simulink model "LSC_Integration"  (R2022b)
settings: Solver=FixedStepDiscrete  StartTime=0.0  StopTime=130  FixedStep=Ts  RelTol=1e-3
values from neighbouring files (symbols this model uses):
  LUX_AHB = 50    [build_B3_AHB.m]
  LUX_OFF = 2000    [build_B2_AutoHeadlamp.m]
  LUX_ON = 1000    [build_B2_AutoHeadlamp.m]
  T_OFF = 5    [build_B2_AutoHeadlamp.m]
  T_ON = 2    [build_B2_AutoHeadlamp.m]
  T_REARM = 2    [build_B3_AHB.m]
  T_TUNNEL = 0.3    [build_B2_AutoHeadlamp.m]
  Ts = 0.01    [build_B2_AutoHeadlamp.m]    (also in build_B3_AHB.m)
  V_AHB_OFF = 30    [build_B3_AHB.m]
  V_AHB_ON = 40    [build_B3_AHB.m]
undefined symbols (not defined in the file or in its folder): A_ESS_OFF, A_ESS_ON, F_BLINK, F_ESS, F_HYPER, I_NOM, LUX_MAX, N_COMFORT, POS_DIM, R_OPEN, R_SHORT, T_ABSENT, T_ARM, T_CONF, T_DEB, T_FMH, T_FMH_MAX, T_FMH_STEP, T_HEAL, T_INRUSH, T_RECOVER, T_SHORT, T_SOFT, TAIL_DIM, TAU_LUX, U_BAT_MIN, V_EFF, V_ESS, V_RESUME
libraries: simulink x1
settings Model: Creator=LENOVO  LastModifiedBy=LENOVO

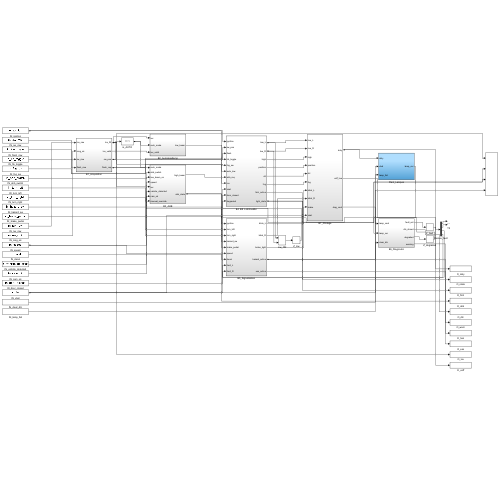
[thumbnail: Simulink's stored preview of the top-level diagram]
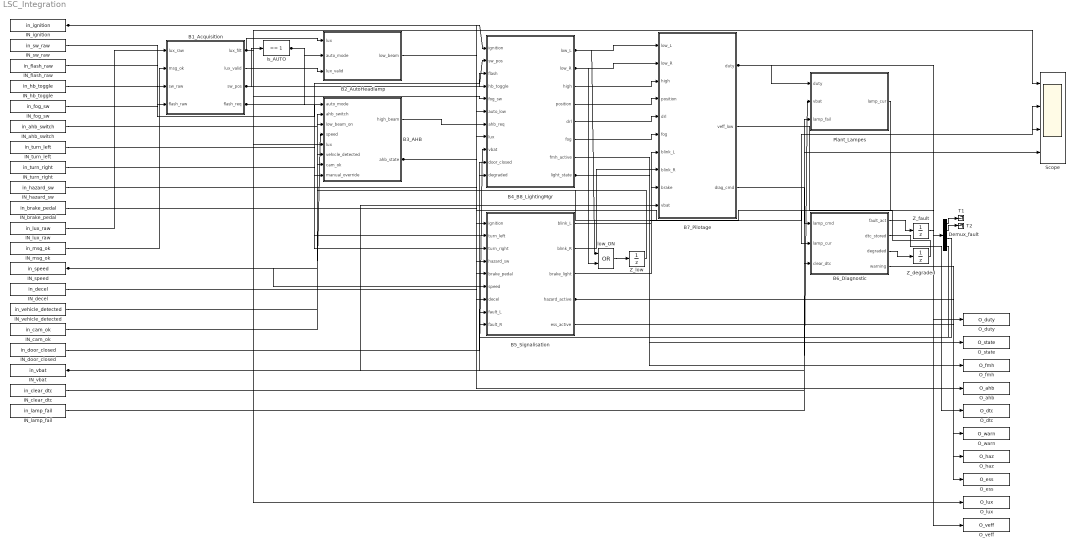
== system LSC_Integration ==
  B1_Acquisition : Subsystem
  B2_AutoHeadlamp : Subsystem
  B3_AHB : Subsystem
  B4_B8_LightingMgr : Subsystem
  B5_Signalisation : Subsystem
  B6_Diagnostic : Subsystem
  B7_Pilotage : Subsystem
  Demux_fault : Demux
  IN_ahb_switch : FromWorkspace  VariableName=in_ahb_switch  SampleTime=Ts  Interpolate=off  OutputAfterFinalValue=Holding final value
  IN_brake_pedal : FromWorkspace  VariableName=in_brake_pedal  SampleTime=Ts  Interpolate=off  OutputAfterFinalValue=Holding final value
  IN_cam_ok : FromWorkspace  VariableName=in_cam_ok  SampleTime=Ts  Interpolate=off  OutputAfterFinalValue=Holding final value
  IN_clear_dtc : FromWorkspace  VariableName=in_clear_dtc  SampleTime=Ts  Interpolate=off  OutputAfterFinalValue=Holding final value
  IN_decel : FromWorkspace  VariableName=in_decel  SampleTime=Ts  OutputAfterFinalValue=Holding final value
  IN_door_closed : FromWorkspace  VariableName=in_door_closed  SampleTime=Ts  Interpolate=off  OutputAfterFinalValue=Holding final value
  IN_flash_raw : FromWorkspace  VariableName=in_flash_raw  SampleTime=Ts  Interpolate=off  OutputAfterFinalValue=Holding final value
  IN_fog_sw : FromWorkspace  VariableName=in_fog_sw  SampleTime=Ts  Interpolate=off  OutputAfterFinalValue=Holding final value
  IN_hazard_sw : FromWorkspace  VariableName=in_hazard_sw  SampleTime=Ts  Interpolate=off  OutputAfterFinalValue=Holding final value
  IN_hb_toggle : FromWorkspace  VariableName=in_hb_toggle  SampleTime=Ts  Interpolate=off  OutputAfterFinalValue=Holding final value
  IN_ignition : FromWorkspace  VariableName=in_ignition  SampleTime=Ts  Interpolate=off  OutputAfterFinalValue=Holding final value
  IN_lamp_fail : FromWorkspace  VariableName=in_lamp_fail  SampleTime=Ts  Interpolate=off  OutputAfterFinalValue=Holding final value
  IN_lux_raw : FromWorkspace  VariableName=in_lux_raw  SampleTime=Ts  OutputAfterFinalValue=Holding final value
  IN_msg_ok : FromWorkspace  VariableName=in_msg_ok  SampleTime=Ts  Interpolate=off  OutputAfterFinalValue=Holding final value
  IN_speed : FromWorkspace  VariableName=in_speed  SampleTime=Ts  OutputAfterFinalValue=Holding final value
  IN_sw_raw : FromWorkspace  VariableName=in_sw_raw  SampleTime=Ts  Interpolate=off  OutputAfterFinalValue=Holding final value
  IN_turn_left : FromWorkspace  VariableName=in_turn_left  SampleTime=Ts  Interpolate=off  OutputAfterFinalValue=Holding final value
  IN_turn_right : FromWorkspace  VariableName=in_turn_right  SampleTime=Ts  Interpolate=off  OutputAfterFinalValue=Holding final value
  IN_vbat : FromWorkspace  VariableName=in_vbat  SampleTime=Ts  OutputAfterFinalValue=Holding final value
  IN_vehicle_detected : FromWorkspace  VariableName=in_vehicle_detected  SampleTime=Ts  Interpolate=off  OutputAfterFinalValue=Holding final value
  O_ahb : ToWorkspace  VariableName=O_ahb  SaveFormat=Timeseries  SampleTime=-1
  O_dtc : ToWorkspace  VariableName=O_dtc  SaveFormat=Timeseries  SampleTime=-1
  O_duty : ToWorkspace  VariableName=O_duty  SaveFormat=Timeseries  SampleTime=-1
  O_ess : ToWorkspace  VariableName=O_ess  SaveFormat=Timeseries  SampleTime=-1
  O_fmh : ToWorkspace  VariableName=O_fmh  SaveFormat=Timeseries  SampleTime=-1
  O_haz : ToWorkspace  VariableName=O_haz  SaveFormat=Timeseries  SampleTime=-1
  O_lux : ToWorkspace  VariableName=O_lux  SaveFormat=Timeseries  SampleTime=-1
  O_state : ToWorkspace  VariableName=O_state  SaveFormat=Timeseries  SampleTime=-1
  O_veff : ToWorkspace  VariableName=O_veff  SaveFormat=Timeseries  SampleTime=-1
  O_warn : ToWorkspace  VariableName=O_warn  SaveFormat=Timeseries  SampleTime=-1
  Plant_Lampes : Subsystem
  Scope : Scope  NumInputPorts=4
  T1 : Terminator
  T2 : Terminator
  Z_degraded : UnitDelay  SampleTime=Ts  HasFrameUpgradeWarning=on
  Z_fault : UnitDelay  SampleTime=Ts  HasFrameUpgradeWarning=on
  Z_low : UnitDelay  SampleTime=Ts  HasFrameUpgradeWarning=on
  is_AUTO : simulink/Logic and Bit Operations/Compare To Constant  relop===  const=1  OutDataTypeStr=boolean
  low_ON : Logic  Operator=OR  AllPortsSameDT=off  OutDataTypeStr=boolean
  wires:
  IN_lux_raw/1 -> B1_Acquisition/1(lux_raw)
  IN_msg_ok/1 -> B1_Acquisition/2(msg_ok)
  IN_sw_raw/1 -> B1_Acquisition/3(sw_raw)
  IN_flash_raw/1 -> B1_Acquisition/4(flash_raw)
  B1_Acquisition/3(sw_pos) -> is_AUTO/1, B4_B8_LightingMgr/2(sw_pos)
  B1_Acquisition/1(lux_filt) -> B2_AutoHeadlamp/1(lux), B3_AHB/5(lux), B4_B8_LightingMgr/8(lux), O_lux/1, Scope/1
  is_AUTO/1 -> B2_AutoHeadlamp/2(auto_mode), B3_AHB/1(auto_mode)
  B1_Acquisition/2(lux_valid) -> B2_AutoHeadlamp/3(lux_valid)
  IN_ahb_switch/1 -> B3_AHB/2(ahb_switch)
  Z_low/1 -> B3_AHB/3(low_beam_on)
  IN_speed/1 -> B3_AHB/4(speed), B5_Signalisation/6(speed)
  IN_vehicle_detected/1 -> B3_AHB/6(vehicle_detected)
  IN_cam_ok/1 -> B3_AHB/7(cam_ok)
  B1_Acquisition/4(flash_req) -> B3_AHB/8(manual_override), B4_B8_LightingMgr/3(flash)
  IN_ignition/1 -> B4_B8_LightingMgr/1(ignition), B5_Signalisation/1(ignition)
  IN_hb_toggle/1 -> B4_B8_LightingMgr/4(hb_toggle)
  IN_fog_sw/1 -> B4_B8_LightingMgr/5(fog_sw)
  B2_AutoHeadlamp/1(low_beam) -> B4_B8_LightingMgr/6(auto_low)
  B3_AHB/1(high_beam) -> B4_B8_LightingMgr/7(ahb_req)
  IN_vbat/1 -> B4_B8_LightingMgr/9(vbat), B7_Pilotage/10(vbat), Plant_Lampes/2(vbat)
  IN_door_closed/1 -> B4_B8_LightingMgr/10(door_closed)
  Z_degraded/1 -> B4_B8_LightingMgr/11(degraded)
  B4_B8_LightingMgr/1(low_L) -> low_ON/1, B7_Pilotage/1(low_L)
  B4_B8_LightingMgr/2(low_R) -> low_ON/2, B7_Pilotage/2(low_R)
  low_ON/1 -> Z_low/1
  IN_turn_left/1 -> B5_Signalisation/2(turn_left)
  IN_turn_right/1 -> B5_Signalisation/3(turn_right)
  IN_hazard_sw/1 -> B5_Signalisation/4(hazard_sw)
  IN_brake_pedal/1 -> B5_Signalisation/5(brake_pedal)
  IN_decel/1 -> B5_Signalisation/7(decel)
  Demux_fault/3 -> B5_Signalisation/8(fault_L)
  Demux_fault/4 -> B5_Signalisation/9(fault_R)
  Demux_fault/1 -> T1/1
  Demux_fault/2 -> T2/1
  B4_B8_LightingMgr/3(high) -> B7_Pilotage/3(high)
  B4_B8_LightingMgr/4(position) -> B7_Pilotage/4(position)
  B4_B8_LightingMgr/5(drl) -> B7_Pilotage/5(drl)
  B4_B8_LightingMgr/6(fog) -> B7_Pilotage/6(fog)
  B5_Signalisation/1(blink_L) -> B7_Pilotage/7(blink_L)
  B5_Signalisation/2(blink_R) -> B7_Pilotage/8(blink_R)
  B5_Signalisation/3(brake_light) -> B7_Pilotage/9(brake)
  B7_Pilotage/1(duty) -> Plant_Lampes/1(duty), O_duty/1
  IN_lamp_fail/1 -> Plant_Lampes/3(lamp_fail)
  B7_Pilotage/3(diag_cmd) -> B6_Diagnostic/1(lamp_cmd)
  Plant_Lampes/1(lamp_cur) -> B6_Diagnostic/2(lamp_cur)
  IN_clear_dtc/1 -> B6_Diagnostic/3(clear_dtc)
  B6_Diagnostic/1(fault_act) -> Z_fault/1
  Z_fault/1 -> Demux_fault/1
  B6_Diagnostic/3(degraded) -> Z_degraded/1
  B4_B8_LightingMgr/8(light_state) -> O_state/1, Scope/2
  B4_B8_LightingMgr/7(fmh_active) -> O_fmh/1
  B3_AHB/2(ahb_state) -> O_ahb/1, Scope/3
  B6_Diagnostic/2(dtc_stored) -> O_dtc/1
  B6_Diagnostic/4(warning) -> O_warn/1
  B5_Signalisation/4(hazard_active) -> O_haz/1, Scope/4
  B5_Signalisation/5(ess_active) -> O_ess/1
  B7_Pilotage/2(veff_low) -> O_veff/1

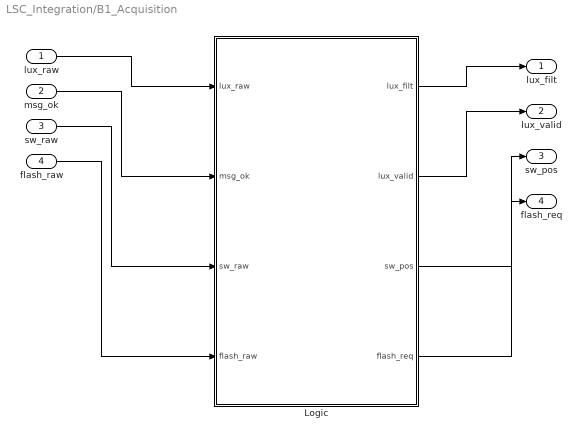
== system LSC_Integration/B1_Acquisition ==
  lux_raw : Inport
  msg_ok : Inport  Port=2
  sw_raw : Inport  Port=3
  flash_raw : Inport  Port=4
  Logic : MATLAB Function  TreatAsAtomicUnit=on
  lux_filt : Outport
  lux_valid : Outport  Port=2
  sw_pos : Outport  Port=3
  flash_req : Outport  Port=4
  wires:
  lux_raw/1 -> Logic/1(lux_raw)
  msg_ok/1 -> Logic/2(msg_ok)
  sw_raw/1 -> Logic/3(sw_raw)
  flash_raw/1 -> Logic/4(flash_raw)
  Logic/1(lux_filt) -> lux_filt/1
  Logic/2(lux_valid) -> lux_valid/1
  Logic/3(sw_pos) -> sw_pos/1
  Logic/4(flash_req) -> flash_req/1

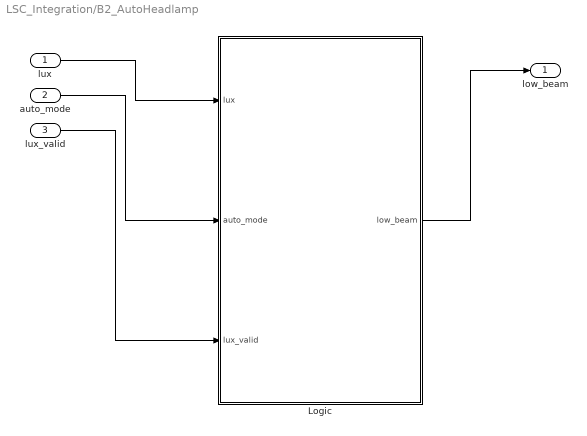
== system LSC_Integration/B2_AutoHeadlamp ==
  lux : Inport
  auto_mode : Inport  Port=2
  lux_valid : Inport  Port=3
  Logic : MATLAB Function  TreatAsAtomicUnit=on
  low_beam : Outport
  wires:
  lux/1 -> Logic/1(lux)
  auto_mode/1 -> Logic/2(auto_mode)
  lux_valid/1 -> Logic/3(lux_valid)
  Logic/1(low_beam) -> low_beam/1

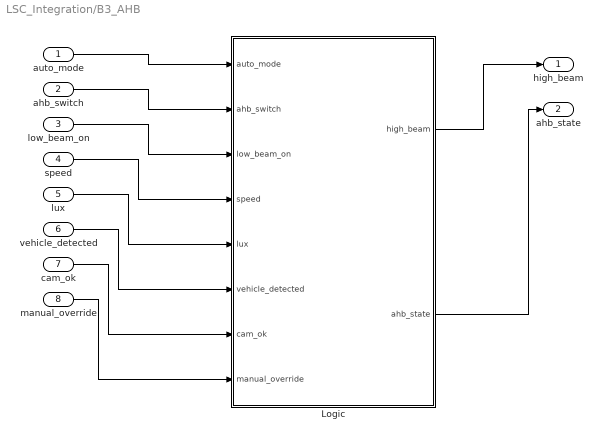
== system LSC_Integration/B3_AHB ==
  auto_mode : Inport
  ahb_switch : Inport  Port=2
  low_beam_on : Inport  Port=3
  speed : Inport  Port=4
  lux : Inport  Port=5
  vehicle_detected : Inport  Port=6
  cam_ok : Inport  Port=7
  manual_override : Inport  Port=8
  Logic : MATLAB Function  TreatAsAtomicUnit=on
  high_beam : Outport
  ahb_state : Outport  Port=2
  wires:
  auto_mode/1 -> Logic/1(auto_mode)
  ahb_switch/1 -> Logic/2(ahb_switch)
  low_beam_on/1 -> Logic/3(low_beam_on)
  speed/1 -> Logic/4(speed)
  lux/1 -> Logic/5(lux)
  vehicle_detected/1 -> Logic/6(vehicle_detected)
  cam_ok/1 -> Logic/7(cam_ok)
  manual_override/1 -> Logic/8(manual_override)
  Logic/1(high_beam) -> high_beam/1
  Logic/2(ahb_state) -> ahb_state/1

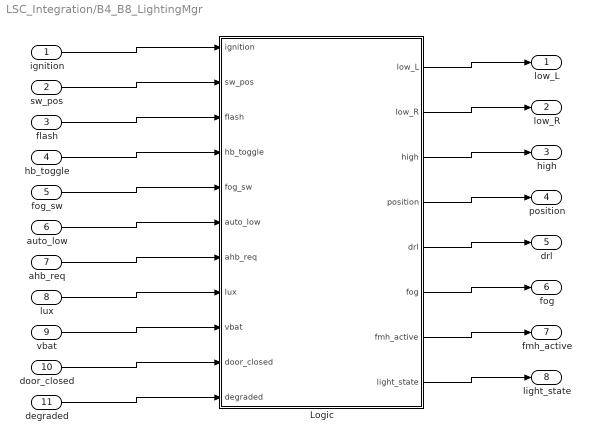
== system LSC_Integration/B4_B8_LightingMgr ==
  ignition : Inport
  sw_pos : Inport  Port=2
  flash : Inport  Port=3
  hb_toggle : Inport  Port=4
  fog_sw : Inport  Port=5
  auto_low : Inport  Port=6
  ahb_req : Inport  Port=7
  lux : Inport  Port=8
  vbat : Inport  Port=9
  door_closed : Inport  Port=10
  degraded : Inport  Port=11
  Logic : MATLAB Function  TreatAsAtomicUnit=on
  low_L : Outport
  low_R : Outport  Port=2
  high : Outport  Port=3
  position : Outport  Port=4
  drl : Outport  Port=5
  fog : Outport  Port=6
  fmh_active : Outport  Port=7
  light_state : Outport  Port=8
  wires:
  ignition/1 -> Logic/1(ignition)
  sw_pos/1 -> Logic/2(sw_pos)
  flash/1 -> Logic/3(flash)
  hb_toggle/1 -> Logic/4(hb_toggle)
  fog_sw/1 -> Logic/5(fog_sw)
  auto_low/1 -> Logic/6(auto_low)
  ahb_req/1 -> Logic/7(ahb_req)
  lux/1 -> Logic/8(lux)
  vbat/1 -> Logic/9(vbat)
  door_closed/1 -> Logic/10(door_closed)
  degraded/1 -> Logic/11(degraded)
  Logic/1(low_L) -> low_L/1
  Logic/2(low_R) -> low_R/1
  Logic/3(high) -> high/1
  Logic/4(position) -> position/1
  Logic/5(drl) -> drl/1
  Logic/6(fog) -> fog/1
  Logic/7(fmh_active) -> fmh_active/1
  Logic/8(light_state) -> light_state/1

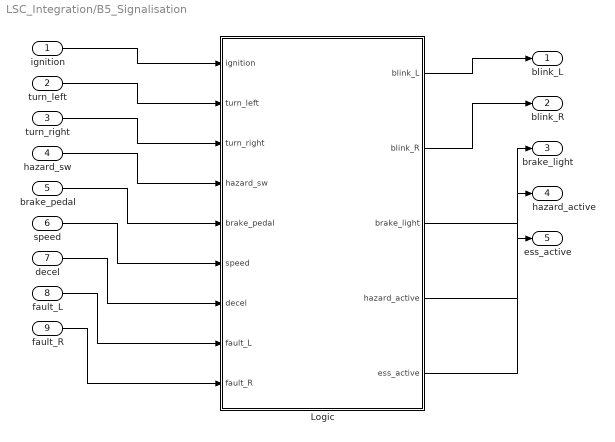
== system LSC_Integration/B5_Signalisation ==
  ignition : Inport
  turn_left : Inport  Port=2
  turn_right : Inport  Port=3
  hazard_sw : Inport  Port=4
  brake_pedal : Inport  Port=5
  speed : Inport  Port=6
  decel : Inport  Port=7
  fault_L : Inport  Port=8
  fault_R : Inport  Port=9
  Logic : MATLAB Function  TreatAsAtomicUnit=on
  blink_L : Outport
  blink_R : Outport  Port=2
  brake_light : Outport  Port=3
  hazard_active : Outport  Port=4
  ess_active : Outport  Port=5
  wires:
  ignition/1 -> Logic/1(ignition)
  turn_left/1 -> Logic/2(turn_left)
  turn_right/1 -> Logic/3(turn_right)
  hazard_sw/1 -> Logic/4(hazard_sw)
  brake_pedal/1 -> Logic/5(brake_pedal)
  speed/1 -> Logic/6(speed)
  decel/1 -> Logic/7(decel)
  fault_L/1 -> Logic/8(fault_L)
  fault_R/1 -> Logic/9(fault_R)
  Logic/1(blink_L) -> blink_L/1
  Logic/2(blink_R) -> blink_R/1
  Logic/3(brake_light) -> brake_light/1
  Logic/4(hazard_active) -> hazard_active/1
  Logic/5(ess_active) -> ess_active/1

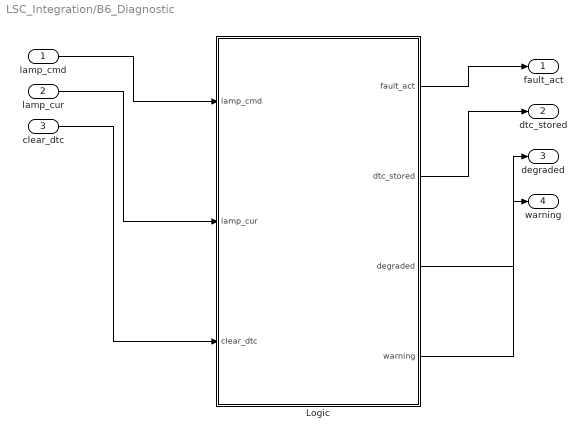
== system LSC_Integration/B6_Diagnostic ==
  lamp_cmd : Inport
  lamp_cur : Inport  Port=2
  clear_dtc : Inport  Port=3
  Logic : MATLAB Function  TreatAsAtomicUnit=on
  fault_act : Outport
  dtc_stored : Outport  Port=2
  degraded : Outport  Port=3
  warning : Outport  Port=4
  wires:
  lamp_cmd/1 -> Logic/1(lamp_cmd)
  lamp_cur/1 -> Logic/2(lamp_cur)
  clear_dtc/1 -> Logic/3(clear_dtc)
  Logic/1(fault_act) -> fault_act/1
  Logic/2(dtc_stored) -> dtc_stored/1
  Logic/3(degraded) -> degraded/1
  Logic/4(warning) -> warning/1

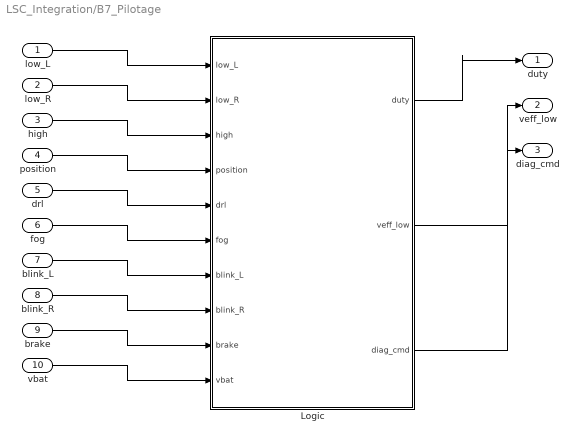
== system LSC_Integration/B7_Pilotage ==
  low_L : Inport
  low_R : Inport  Port=2
  high : Inport  Port=3
  position : Inport  Port=4
  drl : Inport  Port=5
  fog : Inport  Port=6
  blink_L : Inport  Port=7
  blink_R : Inport  Port=8
  brake : Inport  Port=9
  vbat : Inport  Port=10
  Logic : MATLAB Function  TreatAsAtomicUnit=on
  duty : Outport
  veff_low : Outport  Port=2
  diag_cmd : Outport  Port=3
  wires:
  low_L/1 -> Logic/1(low_L)
  low_R/1 -> Logic/2(low_R)
  high/1 -> Logic/3(high)
  position/1 -> Logic/4(position)
  drl/1 -> Logic/5(drl)
  fog/1 -> Logic/6(fog)
  blink_L/1 -> Logic/7(blink_L)
  blink_R/1 -> Logic/8(blink_R)
  brake/1 -> Logic/9(brake)
  vbat/1 -> Logic/10(vbat)
  Logic/1(duty) -> duty/1
  Logic/2(veff_low) -> veff_low/1
  Logic/3(diag_cmd) -> diag_cmd/1

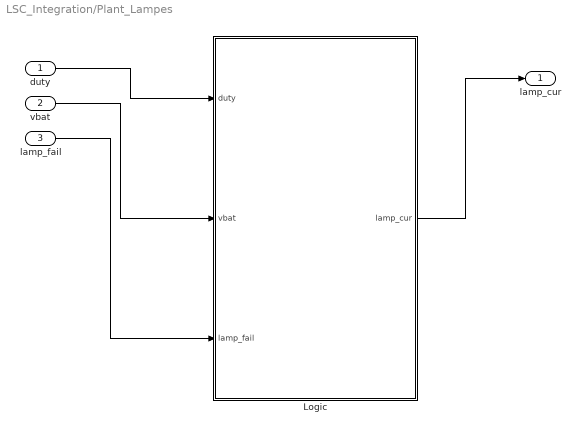
== system LSC_Integration/Plant_Lampes ==
  duty : Inport
  vbat : Inport  Port=2
  lamp_fail : Inport  Port=3
  Logic : MATLAB Function  TreatAsAtomicUnit=on
  lamp_cur : Outport
  wires:
  duty/1 -> Logic/1(duty)
  vbat/1 -> Logic/2(vbat)
  lamp_fail/1 -> Logic/3(lamp_fail)
  Logic/1(lamp_cur) -> lamp_cur/1

== matlab function LSC_Integration/B5_Signalisation/Logic ==
  data: ignition input; blink_L output boolean size=1; turn_left input; turn_right input; hazard_sw input; brake_pedal input; speed input; decel input; fault_L input; fault_R input; blink_R output boolean size=1; brake_light output boolean size=1; hazard_active output boolean size=1; ess_active output boolean size=1; Ts parameter; F_BLINK parameter; F_HYPER parameter; T_SHORT parameter; N_COMFORT parameter; A_ESS_ON parameter; A_ESS_OFF parameter; V_ESS parameter; F_ESS parameter; V_RESUME parameter
function [blink_L, blink_R, brake_light, hazard_active, ess_active] = B5_Signal(ignition, turn_left, turn_right, hazard_sw, brake_pedal, speed, decel, fault_L, fault_R, Ts, F_BLINK, F_HYPER, T_SHORT, N_COMFORT, A_ESS_ON, A_ESS_OFF, V_ESS, F_ESS, V_RESUME)
%#codegen
% B5 - Clignotants, feux de detresse, feux stop et signal de freinage d'urgence (ESS)
% decel : deceleration longitudinale [m/s2], positive quand le vehicule freine
persistent init tside comfort press_t prevL prevR prev_req ph cyc ess ph_ess ess_seen auto_haz
if isempty(init)
    init = true; tside = 0; comfort = false; press_t = 0; prevL = false; prevR = false;
    prev_req = 0; ph = 0; cyc = 0; ess = false; ph_ess = 0; ess_seen = false; auto_haz = false;
end

% ---------- 1) Signal de freinage d'urgence ESS (REQ-LSC-20)
if ~ess && brake_pedal && decel > A_ESS_ON && speed > V_ESS
    ess = true; ph_ess = 0; ess_seen = true;          % freinage d'urgence detecte
elseif ess && (decel < A_ESS_OFF || ~brake_pedal)
    ess = false;                                       % fin du freinage d'urgence
end

% ---------- 2) Feux de detresse automatiques apres arret d'urgence (REQ-LSC-21)
if ess_seen && speed < 0.5
    auto_haz = true; ess_seen = false;
end
if auto_haz && speed > V_RESUME
    auto_haz = false;                                  % le vehicule repart
end
hazard = hazard_sw || auto_haz;

% ---------- 3) Demande de clignotement : 0 aucun, 1 gauche, 2 droite, 3 detresse
if hazard
    req = 3;                                           % detresse prioritaire, meme contact coupe (REQ-LSC-18)
    tside = 0; comfort = false;
elseif ignition
    if turn_left && ~prevL                             % debut d'appui a gauche
        tside = 1; press_t = 0; comfort = false;
    elseif turn_right && ~prevR                        % debut d'appui a droite
        tside = 2; press_t = 0; comfort = false;
    end
    if (tside == 1 && turn_left) || (tside == 2 && turn_right)
        press_t = press_t + Ts;                        % duree d'appui
    end
    if (tside == 1 && ~turn_left && prevL) || (tside == 2 && ~turn_right && prevR)
        if press_t < T_SHORT
            comfort = true;                            % impulsion courte : mode autoroute (REQ-LSC-17)
        else
            tside = 0;                                 % levier relache : arret
        end
    end
    if comfort && cyc >= N_COMFORT
        tside = 0; comfort = false;                    % 3 cycles effectues
    end
    req = tside;
else
    req = 0; tside = 0; comfort = false;
end
prevL = turn_left; prevR = turn_right;

% ---------- 4) Generateur de clignotement (REQ-LSC-16, hyper-clignotement REQ-LSC-23)
if (req == 1 && fault_L) || (req == 2 && fault_R) || (req == 3 && (fault_L || fault_R))
    period = 1 / F_HYPER;                              % lampe grillee : frequence doublee
else
    period = 1 / F_BLINK;
end
if req ~= prev_req
    ph = 0; cyc = 0;                                   % nouvelle demande : on repart d'un flash allume
end
prev_req = req;
on = false;
if req > 0
    on = ph < period / 2;                              % rapport cyclique 50 %
    ph = ph + Ts;
    if ph >= period - 1e-9
        ph = ph - period; cyc = cyc + 1;               % un cycle complet
    end
end
blink_L = on && (req == 1 || req == 3);
blink_R = on && (req == 2 || req == 3);

% ---------- 5) Feux stop (REQ-LSC-19) et clignotement ESS
if ess
    brake_light = ph_ess < 0.5 / F_ESS;
    ph_ess = ph_ess + Ts;
    if ph_ess >= 1 / F_ESS - 1e-9, ph_ess = ph_ess - 1 / F_ESS; end
else
    brake_light = brake_pedal;                         % allumage direct a l'appui
end
hazard_active = hazard;
ess_active = ess;

== matlab function LSC_Integration/B6_Diagnostic/Logic ==
  data: lamp_cmd input; fault_act output boolean size=[4 1]; lamp_cur input; clear_dtc input; dtc_stored output uint16 size=1; degraded output uint8 size=1; warning output boolean size=1; Ts parameter; I_NOM parameter; R_OPEN parameter; R_SHORT parameter; T_INRUSH parameter; T_CONF parameter; T_HEAL parameter
function [fault_act, dtc_stored, degraded, warning] = B6_Diag(lamp_cmd, lamp_cur, clear_dtc, Ts, I_NOM, R_OPEN, R_SHORT, T_INRUSH, T_CONF, T_HEAL)
%#codegen
% B6 - Diagnostic des lampes par mesure du courant
% Lampes : 1 croisement G, 2 croisement D, 3 clignotant G, 4 clignotant D
% dtc_stored : bits 0-3 = circuit ouvert (lampe grillee), bits 4-7 = court-circuit
persistent ton tbo tbs tgood fo fs stored
if isempty(ton)
    ton = zeros(4,1); tbo = zeros(4,1); tbs = zeros(4,1); tgood = zeros(4,1);
    fo = false(4,1); fs = false(4,1); stored = uint16(0);
end
cmd = logical(lamp_cmd(:));  cur = lamp_cur(:);
for i = 1:4
    if cmd(i)
        ton(i) = min(ton(i) + Ts, 100);           % temps depuis l'allumage
    else
        ton(i) = 0;
    end
    if cmd(i) && ton(i) > T_INRUSH + Ts/2         % on ne juge qu'apres le pic d'allumage
        r = cur(i) / I_NOM(i);                    % courant mesure / courant nominal
        bad_open  = r < R_OPEN;                   % < 20 % : lampe grillee (REQ-LSC-22)
        bad_short = r > R_SHORT;                  % > 150 % : court-circuit (REQ-LSC-22)
        if bad_open,  tbo(i) = tbo(i) + Ts; else, tbo(i) = 0; end
        if bad_short, tbs(i) = tbs(i) + Ts; else, tbs(i) = 0; end
        if tbo(i) > T_CONF + Ts/2                 % confirmation 100 ms
            fo(i) = true; stored = bitor(stored, bitshift(uint16(1), i-1));
        end
        if tbs(i) > T_CONF + Ts/2
            fs(i) = true; stored = bitor(stored, bitshift(uint16(1), i+3));
        end
        if ~bad_open && ~bad_short                % mesure correcte : guerison
            tgood(i) = min(tgood(i) + Ts, 100);
            if tgood(i) > T_HEAL + Ts/2
                fo(i) = false; fs(i) = false;     % defaut plus actif (le DTC reste memorise)
            end
        else
            tgood(i) = 0;
        end
    else
        tbo(i) = 0; tbs(i) = 0;                   % lampe eteinte : on ne peut pas juger
    end
end
act = fo | fs;
if clear_dtc                                      % effacement par l'outil de diagnostic
    stored = uint16(0);
    for i = 1:4
        if fo(i), stored = bitor(stored, bitshift(uint16(1), i-1)); end
        if fs(i), stored = bitor(stored, bitshift(uint16(1), i+3)); end
    end
end
fault_act  = act;
dtc_stored = stored;
degraded   = uint8(act(1)) + 2*uint8(act(2));     % 0 aucun, 1 croisement G, 2 croisement D, 3 les deux (REQ-LSC-24)
warning    = any(act);                            % temoin defaut au tableau de bord

== matlab function LSC_Integration/B7_Pilotage/Logic ==
  data: low_L input; duty output uint8 size=[8 1]; low_R input; high input; position input; drl input; fog input; blink_L input; blink_R input; brake input; vbat input; veff_low output double size=1; diag_cmd output boolean size=[4 1]; Ts parameter; V_EFF parameter; T_SOFT parameter; POS_DIM parameter; TAIL_DIM parameter
function [duty, veff_low, diag_cmd] = B7_Driver(low_L, low_R, high, position, drl, fog, blink_L, blink_R, brake, vbat, Ts, V_EFF, T_SOFT, POS_DIM, TAIL_DIM)
%#codegen
% B7 - Pilotage des sorties (PWM)
% duty (8 voies, %) : 1 croisement G, 2 croisement D, 3 route, 4 LED avant DRL/veilleuse,
%                     5 clignotant G, 6 clignotant D, 7 LED arriere stop/position, 8 antibrouillard AR
persistent ramp
if isempty(ramp), ramp = zeros(4,1); end         % rampes : croisement G, croisement D, route, antibrouillard

% 1) Regulation de tension des lampes halogenes : tension efficace constante = V_EFF
d_reg = min(1, (V_EFF / max(vbat, 1))^2);         % Veff = sqrt(duty) * Vbat

% 2) Demarrage progressif (soft-start) : limite le pic de courant du filament froid
req = [low_L; low_R; high; fog];
for i = 1:4
    if req(i)
        ramp(i) = min(ramp(i) + Ts / T_SOFT, 1);  % 0 -> 100 % en T_SOFT
    else
        ramp(i) = 0;                              % extinction immediate
    end
end
d = zeros(8,1);
d(1) = ramp(1) * d_reg;  d(2) = ramp(2) * d_reg;  d(3) = ramp(3) * d_reg;  d(8) = ramp(4) * d_reg;

% 3) LED avant a deux niveaux : DRL plein (100 %), veilleuse attenuee (REQ-LSC-05)
if drl
    d(4) = 1;
elseif position
    d(4) = POS_DIM;
end
% 4) Clignotants : pleine tension regulee des le 1er pas (pas de rampe, flash net)
d(5) = double(blink_L) * d_reg;  d(6) = double(blink_R) * d_reg;
% 5) LED arriere a deux niveaux : stop plein, position attenuee
if brake
    d(7) = 1;
elseif position
    d(7) = TAIL_DIM;
end

duty     = uint8(round(100 * d));
veff_low = sqrt(d(1)) * vbat;                     % tension efficace vue par le croisement gauche
diag_cmd = [d(1) > 0; d(2) > 0; d(5) > 0; d(6) > 0];   % lampes allumees, pour le diagnostic B6

== matlab function LSC_Integration/Plant_Lampes/Logic ==
  data: duty input; lamp_cur output double size=[4 1]; vbat input; lamp_fail input; I_NOM parameter
function lamp_cur = Plant_Lamps(duty, vbat, lamp_fail, I_NOM)
%#codegen
% MODELE DE L'ENVIRONNEMENT (pas du logiciel embarque) : courant moyen consomme par 4 lampes
% lampes surveillees : voie 1 croisement G, 2 croisement D, 5 clignotant G, 6 clignotant D
% lamp_fail : 1 lampe normale, 0 lampe grillee, 2 court-circuit partiel
d = double(duty(:)) / 100;
idx = [1; 2; 5; 6];
lamp_cur = I_NOM(:) .* d(idx) * (vbat / 13.5) .* lamp_fail(:);

== matlab function LSC_Integration/B2_AutoHeadlamp/Logic ==
  data: lux input; low_beam output; auto_mode input; lux_valid input; Ts parameter; LUX_ON parameter; LUX_OFF parameter; T_ON parameter; T_OFF parameter; T_TUNNEL parameter
function low_beam = AutoHeadlampLogic(lux, auto_mode, lux_valid, Ts, LUX_ON, LUX_OFF, T_ON, T_OFF, T_TUNNEL)
%#codegen
% B2 - Auto Headlamp : allumage/extinction automatique avec hysteresis
persistent st cnt buf idx          % memoire conservee d'un pas a l'autre
N = 50;                            % 50 x 10 ms = 0,5 s d'historique
if isempty(st)                     % initialisation au 1er pas
    st = false; cnt = 0; buf = 10000*ones(1, N); idx = 1;
end
% --- Detection tunnel : chute > 80 % en 0,5 s
lux_past = buf(idx);
buf(idx) = lux;
idx = mod(idx, N) + 1;
tunnel = (lux < 0.2*lux_past) && (lux < LUX_ON);

% --- Logique principale
if ~auto_mode
    st = false; cnt = 0;           % pas en AUTO : B2 ne demande rien
elseif ~lux_valid
    st = true;  cnt = 0;           % capteur en defaut : etat sur
elseif ~st                         % feux eteints
    if lux < LUX_ON
        cnt = cnt + Ts;
        if (cnt > T_ON + Ts/2) || (tunnel && cnt > T_TUNNEL + Ts/2)
            st = true; cnt = 0;
        end
    else
        cnt = 0;                   % condition interrompue -> on recommence
    end
else                               % feux allumes
    if lux > LUX_OFF
        cnt = cnt + Ts;
        if cnt > T_OFF + Ts/2
            st = false; cnt = 0;
        end
    else
        cnt = 0;
    end
end
low_beam = st;

== matlab function LSC_Integration/B1_Acquisition/Logic ==
  data: lux_raw input; lux_filt output; msg_ok input; sw_raw input; flash_raw input; lux_valid output; sw_pos output; flash_req output; Ts parameter; TAU_LUX parameter; LUX_MAX parameter; T_ABSENT parameter; T_RECOVER parameter; T_DEB parameter
function [lux_filt, lux_valid, sw_pos, flash_req] = B1_Acquisition(lux_raw, msg_ok, sw_raw, flash_raw, Ts, TAU_LUX, LUX_MAX, T_ABSENT, T_RECOVER, T_DEB)
%#codegen
% B1 - Acquisition et filtrage des entrees
%   lux_raw   : mesure brute du capteur de luminosite [lux]
%   msg_ok    : 1 si le message du capteur est recu a ce pas (bus CAN)
%   sw_raw    : position brute du commodo (0 OFF, 1 AUTO, 2 POSITION, 3 CROISEMENT)
%   flash_raw : contact brut du levier d'appel de phares
persistent init yf valid absent_cnt good_cnt sw_last sw_cnt sw_out fl_last fl_cnt fl_out
if isempty(init)
    init = true; yf = lux_raw; valid = true; absent_cnt = 0; good_cnt = 0;
    sw_last = sw_raw; sw_cnt = 0; sw_out = sw_raw;
    fl_last = flash_raw; fl_cnt = 0; fl_out = flash_raw;
end

% ---------- 1) Diagnostic du capteur de luminosite (REQ-LSC-09)
in_range = (lux_raw >= 0) && (lux_raw <= LUX_MAX);
if msg_ok
    absent_cnt = 0;
else
    absent_cnt = min(absent_cnt + Ts, 100);
end
absent = absent_cnt > T_ABSENT + Ts/2;          % message absent depuis plus de 500 ms
if ~in_range || absent
    valid = false; good_cnt = 0;                % defaut detecte immediatement
elseif msg_ok
    good_cnt = min(good_cnt + Ts, 100);
    if good_cnt > T_RECOVER + Ts/2              % retour a la normale apres 1 s de mesures correctes
        valid = true;
    end
end

% ---------- 2) Filtre passe-bas du 1er ordre (NFR-04), fige si mesure non fiable
if in_range && msg_ok
    if lux_raw < 0.2 * yf                       % chute brutale > 80 % (entree de tunnel) :
        yf = lux_raw;                           % suivi immediat, sinon le filtre retarde B2 (REQ-LSC-08)
    else
        a = Ts / (TAU_LUX + Ts);
        yf = yf + a * (lux_raw - yf);
    end
end

% ---------- 3) Anti-rebond du commodo (NFR-04 / REQ-LSC-02)
if sw_raw ~= sw_last
    sw_last = sw_raw; sw_cnt = 0;               % la position bouge : on recommence
else
    sw_cnt = min(sw_cnt + Ts, 100);
    if sw_cnt > T_DEB - Ts/2
        sw_out = sw_raw;                        % stable depuis 50 ms : on valide
    end
end

% ---------- 4) Anti-rebond de l'appel de phares
if flash_raw ~= fl_last
    fl_last = flash_raw; fl_cnt = 0;
else
    fl_cnt = min(fl_cnt + Ts, 100);
    if fl_cnt > T_DEB - Ts/2
        fl_out = flash_raw;
    end
end

lux_filt  = yf;
lux_valid = valid;
sw_pos    = sw_out;
flash_req = fl_out;

== matlab function LSC_Integration/B3_AHB/Logic ==
  data: auto_mode input; high_beam output boolean size=1; ahb_switch input; low_beam_on input; speed input; lux input; vehicle_detected input; cam_ok input; manual_override input; ahb_state output uint8 size=1; Ts parameter; V_AHB_ON parameter; V_AHB_OFF parameter; LUX_AHB parameter; T_REARM parameter
function [high_beam, ahb_state] = AHB_Logic(auto_mode, ahb_switch, low_beam_on, speed, lux, vehicle_detected, cam_ok, manual_override, Ts, V_AHB_ON, V_AHB_OFF, LUX_AHB, T_REARM)
%#codegen
% B3 - Auto High Beam (AHB) : feux de route automatiques
% ahb_state : 0 = OFF (non disponible), 1 = READY (disponible, route non libre)
%             2 = ACTIVE (feux de route), 3 = PAUSE (action manuelle), 4 = FAULT (camera)
persistent spd_ok clear_cnt hb
if isempty(spd_ok)
    spd_ok = false; clear_cnt = 0; hb = false;
end
% --- Hysteresis de vitesse (REQ-LSC-13) : ON a 40 km/h, OFF sous 30 km/h
if speed >= V_AHB_ON
    spd_ok = true;
elseif speed < V_AHB_OFF
    spd_ok = false;
end
% --- Conditions de disponibilite (REQ-LSC-10)
avail = auto_mode && ahb_switch && low_beam_on && spd_ok && (lux < LUX_AHB);

if ~cam_ok                          % camera en defaut -> etat sur (REQ-LSC-14)
    hb = false; clear_cnt = 0; st = 4;
elseif manual_override              % le conducteur est prioritaire (REQ-LSC-15)
    hb = false; clear_cnt = 0; st = 3;
elseif ~avail                       % conditions non reunies
    hb = false; clear_cnt = 0; st = 0;
elseif vehicle_detected             % usager detecte -> croisement immediat (REQ-LSC-11)
    hb = false; clear_cnt = 0; st = 1;
else                                % route libre : confirmation pendant T_REARM (REQ-LSC-12)
    clear_cnt = min(clear_cnt + Ts, 100);
    if clear_cnt > T_REARM + Ts/2
        hb = true;
    end
    if hb
        st = 2;
    else
        st = 1;
    end
end
high_beam = hb;
ahb_state = uint8(st);

== matlab function LSC_Integration/B4_B8_LightingMgr/Logic ==
  data: ignition input; low_L output boolean size=1; sw_pos input; flash input; hb_toggle input; fog_sw input; auto_low input; ahb_req input; lux input; vbat input; door_closed input; degraded input; low_R output boolean size=1; high output boolean size=1; position output boolean size=1; drl output boolean size=1; fog output boolean size=1; fmh_active output boolean size=1; light_state output uint8 size=1; Ts parameter; LUX_ON parameter; T_FMH parameter; T_ARM parameter; T_FMH_STEP parameter; T_FMH_MAX parameter; U_BAT_MIN parameter
function [low_L, low_R, high, position, drl, fog, fmh_active, light_state] = B4_Manager(ignition, sw_pos, flash, hb_toggle, fog_sw, auto_low, ahb_req, lux, vbat, door_closed, degraded, Ts, LUX_ON, T_FMH, T_ARM, T_FMH_STEP, T_FMH_MAX, U_BAT_MIN)
%#codegen
% B4 - Lighting Manager (arbitrage des feux avant) + B8 - Follow-me-home
% sw_pos : 0 OFF, 1 AUTO, 2 POSITION, 3 CROISEMENT      degraded (B6) : 0 aucun, 1 G, 2 D, 3 les deux
persistent init fmh rem tot t_off hb_man fog_st p_ign p_flash p_hb p_fog p_sw
if isempty(init)
    init = true; fmh = false; rem = 0; tot = 0; t_off = 100; hb_man = false; fog_st = false;
    p_ign = ignition; p_flash = flash; p_hb = hb_toggle; p_fog = fog_sw; p_sw = sw_pos;
end
fl_rise = flash && ~p_flash;   hb_rise = hb_toggle && ~p_hb;   fog_rise = fog_sw && ~p_fog;
bat_ok  = vbat >= U_BAT_MIN;

% =============== B8 : FOLLOW-ME-HOME ===============
if p_ign && ~ignition                                   % le conducteur coupe le contact
    t_off = 0;
    if sw_pos == 1 && lux < LUX_ON && T_FMH > 0 && bat_ok   % activation automatique (REQ-LSC-25, 31)
        fmh = true; tot = T_FMH; rem = T_FMH;
    end
end
if ~ignition, t_off = min(t_off + Ts, 1000); end
if fl_rise && ~ignition && bat_ok && (t_off <= T_ARM || fmh)
    if ~fmh, fmh = true; tot = 0; rem = 0; end          % activation manuelle (REQ-LSC-27)
    tot = min(tot + T_FMH_STEP, T_FMH_MAX);             % prolongation (REQ-LSC-28)
    rem = min(rem + T_FMH_STEP, T_FMH_MAX);
end
if fmh
    if ~door_closed
        rem = tot;                                      % porte ouverte : le compteur repart (REQ-LSC-29)
    else
        rem = rem - Ts;
    end
    if rem <= -Ts/2, fmh = false; end                  % duree ecoulee (compteur passe sous 0) : extinction
end
if (ignition && ~p_ign) || (sw_pos ~= p_sw && (sw_pos == 0 || sw_pos == 2)) || ~bat_ok
    fmh = false;                                        % annulation (REQ-LSC-30)
end

% =============== B4 : ARBITRAGE ===============
if fmh                                                  % REQ-LSC-32 : croisement + position seulement
    low = true; hi = false; pos = true; d = false; hb_man = false; fog_st = false;
elseif ignition
    low = (sw_pos == 3) || (sw_pos == 1 && auto_low);   % manuel ou demande de B2 (REQ-LSC-01, 06)
    pos = low || sw_pos == 2;
    if ~low
        hb_man = false;
    elseif hb_rise
        hb_man = ~hb_man;                               % commutation croisement <-> route (REQ-LSC-02)
    end
    hi = (low && (hb_man || (sw_pos == 1 && ahb_req))) || flash;   % manuel > AHB ; appel de phares (REQ-LSC-03, 15)
    d = ~low && sw_pos ~= 2;                            % DRL (REQ-LSC-05)
else
    low = false; hi = false; d = false; hb_man = false;
    pos = sw_pos == 2;                                  % feux de stationnement contact coupe
end
if ~low
    fog_st = false;                                     % antibrouillard impossible sans croisement (REQ-LSC-04)
elseif fog_rise
    fog_st = ~fog_st;
end

low_L = low && ~(degraded == 1 || degraded == 3);       % lampe en defaut : on coupe sa commande (REQ-LSC-24)
low_R = low && ~(degraded == 2 || degraded == 3);
high = hi;  position = pos;  drl = d;  fog = fog_st && low;  fmh_active = fmh;
if fmh, st = 5; elseif hi, st = 4; elseif low, st = 3; elseif pos, st = 2; elseif d, st = 1; else, st = 0; end
light_state = uint8(st);                                % 0 OFF, 1 DRL, 2 POSITION, 3 CROISEMENT, 4 ROUTE, 5 FMH
p_ign = ignition; p_flash = flash; p_hb = hb_toggle; p_fog = fog_sw; p_sw = sw_pos;
